simulink model "fcw_model"  (R2026b)
settings: Solver=FixedStepDiscrete  StopTime=4  FixedStep=0.01
libraries: simulink x1
settings Model: Creator=Hanane  LastModifiedBy=Hanane

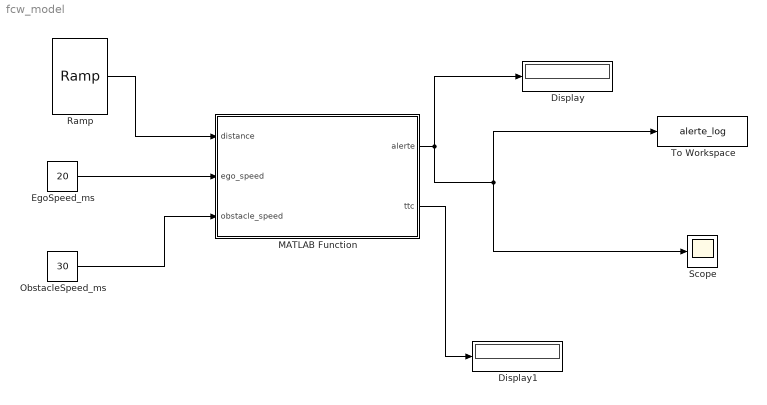
== system fcw_model ==
  Display : Display
  Display1 : Display
  EgoSpeed_ms : Constant  Value=20
  MATLAB Function : MATLAB Function  TreatAsAtomicUnit=on
  ObstacleSpeed_ms : Constant  Value=30
  Ramp : simulink/Sources/Ramp  slope=10  start=0  InitialOutput=50
  Scope : Scope
      settings: ActiveDisplayYMinimum=-0.12499999999999997  ActiveDisplayYMaximum=1.125
  To Workspace : ToWorkspace  VariableName=alerte_log  SaveFormat=Timeseries  SampleTime=-1
  wires:
  EgoSpeed_ms/1 -> MATLAB Function/2(ego_speed)
  ObstacleSpeed_ms/1 -> MATLAB Function/3(obstacle_speed)
  MATLAB Function/1(alerte) -> To Workspace/1, Scope/1, Display/1
  MATLAB Function/2(ttc) -> Display1/1
  Ramp/1 -> MATLAB Function/1(distance)

== matlab function fcw_model/MATLAB Function ==
  data: distance input; alerte output; ego_speed input; obstacle_speed input; ttc output
function [alerte, ttc] = FCW(distance, ego_speed, obstacle_speed)

v_relative = ego_speed - obstacle_speed;

if v_relative <= 1e-6
    ttc = Inf;
else
    ttc = distance / v_relative;
end

alerte = ttc < 4;
end
